simulink library "AFCToolbox2023a"  (R2023a)
settings: Solver=VariableStepAuto  StartTime=0.0  StopTime=10.0  RelTol=1e-3
undefined symbols (not defined in the file or in its folder): AFC5Toolbox_SimuMoudle, AFCToolbox, ax, ay, az, btnSample, C_d, C_dm, C_m, C_t, Control, d, declination_table, dp0, dp1, dp2, dp3, dt, euler_0, g0, I_xyz, inclination_table, J_m, lmd_high, lmd_low, lp_acc_knoise, lp_acc_max, lp_acc_min, lp_acc_seed, lp_GPS_BL_max, lp_GPS_BL_min, lp_GPS_H_max, lp_GPS_H_min, lp_GPS_knoise, lp_GPS_seed, lp_GPS_vel_max, lp_GPS_vel_min, lp_gyro_knoise, lp_gyro_max, lp_gyro_min, lp_gyro_seed, lp_hf_vwind, lp_hs_vwind_interp, lp_kaerorho, lp_kaeroT, lp_kIxyz, lp_kmass, lp_momentx_A0, lp_momentx_Af, lp_momentx_ts, lp_momenty_A0, lp_momenty_Af, lp_momenty_ts, lp_momentz_A0, lp_momentz_Af, lp_momentz_ts, lp_vf_vwind, lp_vs_vwind_interp, lp_vwind_thetax, lp_vwind_thetaz ... (+54)
libraries: $bdroot x104, simulink x75, etargetslib x32, sharedtransform x13, simulink_extras x12, dspstat3 x11, aerolibconvert2 x9, aerolibtransform2 x3, aerolibutil x2, matrix_library x1
(part 5 of 10)

== system AFCToolbox2023a/SimuMoudle/Forces & Moments1/Moments/Disturb ==
  Moment : Inport
  Demux : Demux  Outputs=3
  Dist Mx : Subsystem  mask(Step Disturbe){ts_0=lp_momentx_ts, A0=lp_momentx_A0, Af=lp_momentx_Af}
      mask prompts: ts_0 "Step time (s) :"; A0 "Initial Value (N.m) :"; Af "Final Value (N.m) :"
  Dist My : Subsystem  mask(Step Disturbe){ts_0=lp_momenty_ts, A0=lp_momenty_A0, Af=lp_momenty_Af}
      mask prompts: ts_0 "Step time (s) :"; A0 "Initial Value (N.m) :"; Af "Final Value (N.m) :"
  Dist Mz : Subsystem  mask(Step Disturbe){ts_0=lp_momentz_ts, A0=lp_momentz_A0, Af=lp_momentz_Af}
      mask prompts: ts_0 "Step time (s) :"; A0 "Initial Value (N.m) :"; Af "Final Value (N.m) :"
  Mux : Mux  Inputs=3
  M : Outport
  wires:
  Mux/1 -> M/1
  Moment/1 -> Demux/1
  Demux/1 -> Dist Mx/1(N)
  Demux/2 -> Dist My/1(N)
  Demux/3 -> Dist Mz/1(N)
  Dist Mx/1(D) -> Mux/1
  Dist My/1(D) -> Mux/2
  Dist Mz/1(D) -> Mux/3

== system AFCToolbox2023a/SimuMoudle/Forces & Moments1/Parameters/Air Parameter1 ==
  V : Inport
  h(m) : Inport  Port=2
  Air Model : Subsystem
  Fcn : Fcn  Expr=g0*(6371^2/(6371+u)^2)
  Gain3 : Gain  Gain=0.001
  vel : Scope
  Mach : Outport
  q : Outport  Port=2
  Pressure : Outport  Port=3
  g : Outport  Port=4
  wires:
  Air Model/3(Pressure) -> Pressure/1
  Gain3/1 -> Fcn/1, Air Model/2(h (km))
  Air Model/1(dongYaTou) -> q/1
  Air Model/2(Mach) -> Mach/1
  V/1 -> vel/1, Air Model/1(v)
  h(m)/1 -> Gain3/1
  Fcn/1 -> g/1

== system AFCToolbox2023a/SimuMoudle/Forces & Moments1/Parameters/Inertia Solution ==
  Constant : Constant  Value=I_xyz
  lp_kIxyz : Gain  Gain=lp_kIxyz
  Inertia : Outport
  wires:
  Constant/1 -> lp_kIxyz/1
  lp_kIxyz/1 -> Inertia/1

== system AFCToolbox2023a/SimuMoudle/Forces & Moments1/Parameters/Wind Velocity ==
  height : Inport
  >lp_hf_vwind : Switch  Criteria=u2 > Threshold  Threshold=lp_hf_vwind  SaturateOnIntegerOverflow=off  InputSameDT=off
  Lookup Table h-v wind : Lookup  InputValues=lp_hs_vwind_interp  Table=lp_vs_vwind_interp  SaturateOnIntegerOverflow=off
  Vector : Subsystem
  lp_vf_vwind : Constant  Value=lp_vf_vwind
  lp_vwind_thetax : Constant  Value=lp_vwind_thetax
  lp_vwind_thetaz : Constant  Value=lp_vwind_thetaz
  V Wind : Outport
  wires:
  lp_vf_vwind/1 -> >lp_hf_vwind/1
  height/1 -> Lookup Table h-v wind/1, >lp_hf_vwind/2
  Lookup Table h-v wind/1 -> >lp_hf_vwind/3
  lp_vwind_thetaz/1 -> Vector/2(thetaz)
  lp_vwind_thetax/1 -> Vector/3(thetax)
  Vector/1(xyz) -> V Wind/1
  >lp_hf_vwind/1 -> Vector/1(abs)

== system AFCToolbox2023a/SimuMoudle/Forces & Moments1/Parameters/mass P ==
  Constant 1 : Constant  Value=mass
  lp_kmass : Gain  Gain=lp_kmass
  mass : Outport
  wires:
  lp_kmass/1 -> mass/1
  Constant 1/1 -> lp_kmass/1

== system AFCToolbox2023a/SimuMoudle/Forces & Moments1/Parameters/modulus of vector ==
  vector : Inport
  Divide2 : Product
  Math Function : Math  Operator=sqrt  SignedPower=on
  Sum of Elements : Sum  Inputs=+
  modulus : Outport
  wires:
  Math Function/1 -> modulus/1
  vector/1 -> Divide2/1, Divide2/2
  Divide2/1 -> Sum of Elements/1
  Sum of Elements/1 -> Math Function/1

== system AFCToolbox2023a/SimuMoudle/Position-Control/Consistent formation control /一致性控制——F1 ==
  u0_k : Inport
  X0_k_1 : Inport  Port=2
  X1_k_1 : Inport  Port=3
  X2_k_1 : Inport  Port=4
  dp : Inport  Port=5
  Add{,1..2,4..5,8} (6 alike) : Sum  Inputs=+-
  Add3 : Sum  Inputs=-+
  Add6 : Sum  Inputs=+++
  Add7 : Sum  Inputs=+--
  Bus Selector : BusSelector  OutputSignals=p1_k_1
  Bus Selector1 : BusSelector  OutputSignals=p2_k_1
  Bus Selector2 : BusSelector  OutputSignals=p0_k_1
  Bus Selector3 : BusSelector  OutputSignals=dp1,dp0
  Bus Selector4 : BusSelector  OutputSignals=dp1,dp2
  Bus Selector5 : BusSelector  OutputSignals=v111_k_1
  Bus Selector6 : BusSelector  OutputSignals=v000_k_1
  Demux1 : Demux  Outputs=3
  Gain : Gain  Gain=2
  Gain1 : Gain  Gain=0.5
  Gain2 : Gain  Gain=2
  MATLAB Function1 : MATLAB Function  TreatAsAtomicUnit=on
  MATLAB Function2 : MATLAB Function  TreatAsAtomicUnit=on
  MATLAB Function4 : MATLAB Function  TreatAsAtomicUnit=on
  Mux : Mux  Inputs=3
  Subsystem1 : Subsystem
  X0_k_1_2 : InportShadow  Port=2
  X1_k_1_1 : InportShadow  Port=3
  dp1 : InportShadow  Port=5
  u1_k : Outport
  wires:
  MATLAB Function2/1(result) -> Mux/3
  Demux1/2 -> MATLAB Function1/1(r)
  Demux1/3 -> MATLAB Function2/1(r)
  Demux1/1 -> MATLAB Function4/1(r)
  MATLAB Function1/1(result) -> Mux/2
  MATLAB Function4/1(result) -> Mux/1
  Bus Selector2/1 -> Add/2  "<p0_k_1>"
  dp1/1 -> Bus Selector4/1
  Add8/1 -> u1_k/1
  Gain/1 -> Add6/1
  Add/1 -> Add3/2
  Bus Selector1/1 -> Add1/2  "<p2_k_1>"
  Add5/1 -> Add6/3
  Add2/1 -> Add3/1
  Add4/1 -> Add5/2
  Mux/1 -> Add7/3
  X0_k_1/1 -> Bus Selector6/1
  dp/1 -> Bus Selector3/1
  Subsystem1/1(wxyz) -> Gain/1
  Add1/1 -> Add5/1
  Add7/1 -> Gain2/1
  Bus Selector3/2 -> Add2/2  "<dp0>"
  Bus Selector4/2 -> Add4/2  "<dp2>"
  u0_k/1 -> Add8/1
  Bus Selector3/1 -> Add2/1  "<dp1>"
  X1_k_1/1 -> Bus Selector/1
  Bus Selector6/1 -> Add7/2  "<v000_k_1>"
  Add6/1 -> Gain1/1
  Gain1/1 -> Demux1/1  "控制量z"
  X1_k_1_1/1 -> Bus Selector5/1
  Bus Selector4/1 -> Add4/1  "<dp1>"
  X2_k_1/1 -> Bus Selector1/1
  X0_k_1_2/1 -> Bus Selector2/1
  Bus Selector/1 -> Add1/1, Add/1  "<p1_k_1>"
  Bus Selector5/1 -> Add7/1  "<v111_k_1>"
  Add3/1 -> Add6/2
  Gain2/1 -> Add8/2

== system AFCToolbox2023a/SimuMoudle/Position-Control/Consistent formation control /一致性控制——F2 ==
  dp : Inport
  u0_k : Inport  Port=2
  X0_k_1 : Inport  Port=3
  X1_k_1 : Inport  Port=4
  X2_k_1 : Inport  Port=5
  X3_k_1 : Inport  Port=6
  Add{,1..2,4..5,8} (6 alike) : Sum  Inputs=+-
  Add3 : Sum  Inputs=-+
  Add6 : Sum  Inputs=+++
  Add7 : Sum  Inputs=+--
  Bus Selector : BusSelector  OutputSignals=p1_k_1
  Bus Selector1 : BusSelector  OutputSignals=p2_k_1
  Bus Selector2 : BusSelector  OutputSignals=p2_k_1
  Bus Selector3 : BusSelector  OutputSignals=dp2,dp1
  Bus Selector4 : BusSelector  OutputSignals=dp2,dp3
  Bus Selector5 : BusSelector  OutputSignals=v222_k_1
  Bus Selector6 : BusSelector  OutputSignals=v000_k_1
  Bus Selector7 : BusSelector  OutputSignals=p3_k_1
  Demux1 : Demux  Outputs=3
  Gain : Gain  Gain=2
  Gain1 : Gain  Gain=0.5
  Gain2 : Gain  Gain=2
  MATLAB Function1 : MATLAB Function  TreatAsAtomicUnit=on
  MATLAB Function2 : MATLAB Function  TreatAsAtomicUnit=on
  MATLAB Function3 : MATLAB Function  TreatAsAtomicUnit=on
  Mux : Mux  Inputs=3
  Subsystem2 : Subsystem
  X2_k_1_2 : InportShadow  Port=5
  X2_k_1_3 : InportShadow  Port=5
  dp1 : InportShadow
  u2_k : Outport
  wires:
  MATLAB Function2/1(result) -> Mux/3
  MATLAB Function1/1(result) -> Mux/2
  MATLAB Function3/1(result) -> Mux/1
  Demux1/3 -> MATLAB Function2/1(r)
  Demux1/2 -> MATLAB Function1/1(r)
  Demux1/1 -> MATLAB Function3/1(r)
  Bus Selector4/2 -> Add4/2  "<dp3>"
  Bus Selector3/1 -> Add2/1  "<dp2>"
  Bus Selector7/1 -> Add1/2  "<p3_k_1>"
  X3_k_1/1 -> Bus Selector7/1
  X2_k_1_2/1 -> Bus Selector2/1
  Bus Selector2/1 -> Add1/1  "<p2_k_1>"
  Bus Selector/1 -> Add/2  "<p1_k_1>"
  Bus Selector1/1 -> Add/1  "<p2_k_1>"
  Gain2/1 -> Add8/2
  Add3/1 -> Add6/2
  Bus Selector5/1 -> Add7/1  "<v222_k_1>"
  X2_k_1/1 -> Bus Selector1/1
  Bus Selector4/1 -> Add4/1  "<dp2>"
  X2_k_1_3/1 -> Bus Selector5/1
  Gain1/1 -> Demux1/1  "控制量z"
  Add6/1 -> Gain1/1
  Bus Selector6/1 -> Add7/2  "<v000_k_1>"
  X1_k_1/1 -> Bus Selector/1
  u0_k/1 -> Add8/1
  Bus Selector3/2 -> Add2/2  "<dp1>"
  Add7/1 -> Gain2/1
  Add1/1 -> Add5/1
  Subsystem2/1(wxyz) -> Gain/1
  dp/1 -> Bus Selector3/1
  X0_k_1/1 -> Bus Selector6/1
  Mux/1 -> Add7/3
  Add4/1 -> Add5/2
  Add2/1 -> Add3/1
  Add5/1 -> Add6/3
  Add/1 -> Add3/2
  Gain/1 -> Add6/1
  Add8/1 -> u2_k/1
  dp1/1 -> Bus Selector4/1

== system AFCToolbox2023a/SimuMoudle/Position-Control/Consistent formation control /一致性控制——F3 ==
  dp : Inport
  u0_k : Inport  Port=2
  X0_k_1 : Inport  Port=3
  X1_k_1 : Inport  Port=4
  X2_k_1 : Inport  Port=5
  X3_k_1 : Inport  Port=6
  Add{,1..2,4..5,8} (6 alike) : Sum  Inputs=+-
  Add3 : Sum  Inputs=-+
  Add6 : Sum  Inputs=+++
  Add7 : Sum  Inputs=+--
  Bus Selector : BusSelector  OutputSignals=p2_k_1
  Bus Selector1 : BusSelector  OutputSignals=p3_k_1
  Bus Selector2 : BusSelector  OutputSignals=p3_k_1
  Bus Selector3 : BusSelector  OutputSignals=dp3,dp2
  Bus Selector4 : BusSelector  OutputSignals=dp3,dp1
  Bus Selector5 : BusSelector  OutputSignals=v333_k_1
  Bus Selector6 : BusSelector  OutputSignals=v000_k_1
  Bus Selector7 : BusSelector  OutputSignals=p1_k_1
  Demux1 : Demux  Outputs=3
  Gain : Gain  Gain=2
  Gain1 : Gain  Gain=0.5
  Gain2 : Gain  Gain=2
  MATLAB Function1 : MATLAB Function  TreatAsAtomicUnit=on
  MATLAB Function2 : MATLAB Function  TreatAsAtomicUnit=on
  MATLAB Function3 : MATLAB Function  TreatAsAtomicUnit=on
  Mux : Mux  Inputs=3
  Subsystem1 : Subsystem
  X3_k_1_2 : InportShadow  Port=6
  X3_k_1_3 : InportShadow  Port=6
  dp1 : InportShadow
  u3_k : Outport
  wires:
  MATLAB Function2/1(result) -> Mux/3
  Demux1/2 -> MATLAB Function1/1(r)
  Demux1/3 -> MATLAB Function2/1(r)
  Demux1/1 -> MATLAB Function3/1(r)
  MATLAB Function1/1(result) -> Mux/2
  MATLAB Function3/1(result) -> Mux/1
  Subsystem1/1(wxyz) -> Gain/1
  Bus Selector4/2 -> Add4/2  "<dp1>"
  Bus Selector4/1 -> Add4/1  "<dp3>"
  Bus Selector3/2 -> Add2/2  "<dp2>"
  Bus Selector3/1 -> Add2/1  "<dp3>"
  X1_k_1/1 -> Bus Selector7/1
  X2_k_1/1 -> Bus Selector/1
  X3_k_1/1 -> Bus Selector1/1
  dp1/1 -> Bus Selector4/1
  Add8/1 -> u3_k/1
  Gain/1 -> Add6/1
  Add/1 -> Add3/2
  Add5/1 -> Add6/3
  Add2/1 -> Add3/1
  Add4/1 -> Add5/2
  Mux/1 -> Add7/3
  X0_k_1/1 -> Bus Selector6/1
  dp/1 -> Bus Selector3/1
  Add1/1 -> Add5/1
  Add7/1 -> Gain2/1
  u0_k/1 -> Add8/1
  Bus Selector6/1 -> Add7/2  "<v000_k_1>"
  Add6/1 -> Gain1/1
  Gain1/1 -> Demux1/1  "控制量z"
  X3_k_1_3/1 -> Bus Selector5/1
  Bus Selector5/1 -> Add7/1  "<v333_k_1>"
  Add3/1 -> Add6/2
  Gain2/1 -> Add8/2
  Bus Selector1/1 -> Add/1  "<p3_k_1>"
  Bus Selector/1 -> Add/2  "<p2_k_1>"
  Bus Selector2/1 -> Add1/1  "<p3_k_1>"
  X3_k_1_2/1 -> Bus Selector2/1
  Bus Selector7/1 -> Add1/2  "<p1_k_1>"

== system AFCToolbox2023a/SimuMoudle/Position-Control/Leader/Subsystem ==
  Follower1 : Subsystem
  Follower2 : Subsystem
  Follower3 : Subsystem
  tag scope: X1_k_1=global, X2_k_1=global, X3_k_1=global
  wires:
  Follower3/1(p3_k) -> [p3_k]
  Follower3/4(w3_k) -> [w3_k]
  Follower1/3(v1_k) -> [v1_k]
  Follower2/4(w2_k) -> [w2_k]
  Follower1/1(p1_k) -> [p1_k]
  Follower1/2(X1_k_1) -> [X1_k_1]
  [u] -> Follower3/2(u3_k), Follower2/2(u2_k), Follower1/2(u1_k)
  Follower3/3(v3_k) -> [v3_k]
  Follower1/4(w1_k) -> [w1_k]
  Follower1/5(W1_k) -> [W1_k]
  Follower3/5(W3_k) -> [W3_k]
  Follower2/5(W2_k) -> [W2_k]
  Follower2/3(v2_k) -> [v2_k]
  Follower2/2(X2_k_1) -> [X2_k_1]
  Follower2/1(p2_k) -> [p2_k]
  Follower3/2(X3_k_1) -> [X3_k_1]
  [X0_k_1] -> Follower1/1(X0_k_1), Follower2/1(X0_k_1), Follower3/1(X0_k_1)

== system AFCToolbox2023a/SimuMoudle/Position-Control/Leader/W0-Φ ==
  Digital Clock : DigitalClock  SampleTime=dt
  Gain1 : Gain  Gain=0.2
  Gain2 : Gain  Gain=0.1
  Sin : Trigonometry  Operator=cos
  W0 : Outport
  wires:
  Gain2/1 -> W0/1
  Sin/1 -> Gain2/1
  Gain1/1 -> Sin/1
  Digital Clock/1 -> Gain1/1

== system AFCToolbox2023a/SimuMoudle/Position-Control/Leader/r0-v ==
  Digital Clock : DigitalClock  SampleTime=dt
  Gain1 : Gain  Gain=0.4
  Gain2 : Gain  Gain=0.1
  Scope : Scope
  Sin : Trigonometry
  r0 : Outport
  wires:
  Gain2/1 -> r0/1, Scope/1
  Sin/1 -> Gain2/1
  Gain1/1 -> Sin/1
  Digital Clock/1 -> Gain1/1

== system AFCToolbox2023a/SimuMoudle/Position-Control/Leader/w0-θ ==
  Digital Clock : DigitalClock  SampleTime=dt
  Gain1 : Gain  Gain=0.2
  Gain2 : Gain  Gain=0.1
  Sin : Trigonometry  Operator=cos
  w0 : Outport
  wires:
  Digital Clock/1 -> Gain1/1
  Gain1/1 -> Sin/1
  Sin/1 -> Gain2/1
  Gain2/1 -> w0/1

== system AFCToolbox2023a/SimuMoudle/Position-Control/Leader/质心运动方程 ==
  theta0 : Inport
  phi0 : Inport  Port=2
  v0 : Inport  Port=3
  Cos : Trigonometry  Operator=cos
  Cos1 : Trigonometry  Operator=cos
  Mux : Mux  Inputs=3
  Product : Product  Inputs=3
  Product1 : Product  Inputs=3
  Product2 : Product
  Sin : Trigonometry
  Sin1 : Trigonometry
  v000 : Outport
  wires:
  Sin1/1 -> Product2/1
  Mux/1 -> v000/1
  Product2/1 -> Mux/3
  Cos1/1 -> Product/2, Product1/2
  Sin/1 -> Product1/1
  Product1/1 -> Mux/2
  Product/1 -> Mux/1
  v0/1 -> Product/3, Product1/3, Product2/2
  Cos/1 -> Product/1
  phi0/1 -> Cos1/1, Sin1/1
  theta0/1 -> Sin/1, Cos/1

== system AFCToolbox2023a/SimuMoudle/SimuBaro/Baro model/bias & noise z ==
  normal : Inport
  Sum1 : Sum  Inputs=|++
  Uniform Random Number : UniformRandomNumber  Minimum=noise_min  Maximum=noise_max  Seed=noise_seed  SampleTime=lp_GPS_sample_time
  noise_k : Gain  Gain=noise_k
  real : Outport
  wires:
  noise_k/1 -> Sum1/2
  Uniform Random Number/1 -> noise_k/1
  normal/1 -> Sum1/1
  Sum1/1 -> real/1

== system AFCToolbox2023a/SimuMoudle/SimuGps/LLA model/Subsystem1 ==
  note: 北天东
  note: B:纬度
      | L:经度
      | lat:纬度
      | lon:经度
  X : Inport
  Y : Inport  Port=2
  Z : Inport  Port=3
  Angle Conversion1 : aerolibconvert2/Angle Conversion  IU=rad  OU=deg
  Angle Conversion2 : aerolibconvert2/Angle Conversion  IU=rad  OU=deg
  Bus Creator : BusCreator  Inputs=3
  Bus Creator1 : BusCreator  Inputs=3
  Display5 : Display
  ECEF地心坐标系-经纬高 : MATLAB Function  TreatAsAtomicUnit=on
  LLA2NED : Subsystem
  Mux1 : Mux  Inputs=3
  Mux2 : Mux  Inputs=3
  Mux4 : Mux  Inputs=3
  Scope : Scope
  Scope1 : Scope
  Scope2 : Scope  NumInputPorts=2
  command word1 : Constant  Value=1.978927027963337
  command word10 : Constant  Value=0.402497166193948
  command word11 : Constant  Value=500
  command word3 : Constant  Value=0.402497166193948
  command word4 : Constant  Value=500
  command word9 : Constant  Value=1.978927027963337
  北天东-ECEF地心坐标系 : MATLAB Function  TreatAsAtomicUnit=on
  LLA : Outport
  wires:
  Mux2/1 -> LLA/1
  [lbn] -> LLA2NED/2(LLA)
  X/1 -> Mux4/1, 北天东-ECEF地心坐标系/1(pn)
  Angle Conversion1/1 -> Bus Creator/2  "lat"
  Angle Conversion2/1 -> Bus Creator/1  "lon"
  Mux4/1 -> Scope2/1
  ECEF地心坐标系-经纬高/2(b) -> Bus Creator1/1, Mux2/1  "lat"
  command word9/1 -> Angle Conversion2/1  "lon"
  ECEF地心坐标系-经纬高/1(l) -> Bus Creator1/2, Mux2/2  "lon"
  Bus Creator/1 -> LLA2NED/1(LLA0)
  Bus Creator1/1 -> [lbn], Display5/1, Scope1/1
  LLA2NED/1("sensorout ") -> Scope2/2
  ECEF地心坐标系-经纬高/3(h) -> Bus Creator1/3, Mux2/3  "alt"
  command word10/1 -> Angle Conversion1/1  "lat"
  command word11/1 -> Bus Creator/3  "alt"
  Z/1 -> Mux4/3, 北天东-ECEF地心坐标系/3(pe)
  Y/1 -> Mux4/2, 北天东-ECEF地心坐标系/2(ph)
  Mux1/1 -> Scope/1
  command word4/1 -> 北天东-ECEF地心坐标系/6(Alt0)
  command word3/1 -> 北天东-ECEF地心坐标系/5(Lat0)
  command word1/1 -> 北天东-ECEF地心坐标系/4(Lon0)
  北天东-ECEF地心坐标系/3(DZ) -> ECEF地心坐标系-经纬高/3(z), Mux1/3
  北天东-ECEF地心坐标系/2(DY) -> ECEF地心坐标系-经纬高/2(y), Mux1/2
  北天东-ECEF地心坐标系/1(DX) -> ECEF地心坐标系-经纬高/1(x), Mux1/1

== system AFCToolbox2023a/SimuMoudle/SimuGps/LLA model/bias & noise x ==
  normal : Inport
  Sum1 : Sum  Inputs=|++
  Uniform Random Number : UniformRandomNumber  Minimum=noise_min  Maximum=noise_max  Seed=noise_seed  SampleTime=lp_GPS_sample_time
  noise_k : Gain  Gain=noise_k
  real : Outport
  wires:
  Sum1/1 -> real/1
  normal/1 -> Sum1/1
  Uniform Random Number/1 -> noise_k/1
  noise_k/1 -> Sum1/2

== system AFCToolbox2023a/SimuMoudle/SimuGps/LLA model/bias & noise x2 ==
  normal : Inport
  Sum1 : Sum  Inputs=|++
  Uniform Random Number : UniformRandomNumber  Minimum=noise_min  Maximum=noise_max  Seed=noise_seed  SampleTime=lp_GPS_sample_time
  noise_k : Gain  Gain=noise_k
  real : Outport
  wires:
  noise_k/1 -> Sum1/2
  Uniform Random Number/1 -> noise_k/1
  normal/1 -> Sum1/1
  Sum1/1 -> real/1

== system AFCToolbox2023a/SimuMoudle/SimuGps/LLA model/bias & noise z ==
  normal : Inport
  Sum1 : Sum  Inputs=|++
  Uniform Random Number : UniformRandomNumber  Minimum=noise_min  Maximum=noise_max  Seed=noise_seed  SampleTime=lp_GPS_sample_time
  noise_k : Gain  Gain=noise_k
  real : Outport
  wires:
  Sum1/1 -> real/1
  normal/1 -> Sum1/1
  Uniform Random Number/1 -> noise_k/1
  noise_k/1 -> Sum1/2

== system AFCToolbox2023a/SimuMoudle/SimuGps/Vel model/bias & noise x ==
  normal : Inport
  Sum1 : Sum  Inputs=|++
  Uniform Random Number : UniformRandomNumber  Minimum=noise_min  Maximum=noise_max  Seed=noise_seed  SampleTime=lp_GPS_sample_time
  noise_k : Gain  Gain=noise_k
  real : Outport
  wires:
  noise_k/1 -> Sum1/2
  Uniform Random Number/1 -> noise_k/1
  normal/1 -> Sum1/1
  Sum1/1 -> real/1

== system AFCToolbox2023a/SimuMoudle/SimuGps/Vel model/bias & noise x1 ==
  normal : Inport
  Sum1 : Sum  Inputs=|++
  Uniform Random Number : UniformRandomNumber  Minimum=noise_min  Maximum=noise_max  Seed=noise_seed  SampleTime=lp_GPS_sample_time
  noise_k : Gain  Gain=noise_k
  real : Outport
  wires:
  noise_k/1 -> Sum1/2
  Uniform Random Number/1 -> noise_k/1
  normal/1 -> Sum1/1
  Sum1/1 -> real/1

== system AFCToolbox2023a/SimuMoudle/SimuGps/Vel model/bias & noise x3 ==
  normal : Inport
  Sum1 : Sum  Inputs=|++
  Uniform Random Number : UniformRandomNumber  Minimum=noise_min  Maximum=noise_max  Seed=noise_seed  SampleTime=lp_GPS_sample_time
  noise_k : Gain  Gain=noise_k
  real : Outport
  wires:
  Sum1/1 -> real/1
  normal/1 -> Sum1/1
  Uniform Random Number/1 -> noise_k/1
  noise_k/1 -> Sum1/2

== system AFCToolbox2023a/SimuMoudle/SimuICM/acclerate  model2/Subsystem ==
  normal : Inport
  Add4 : Sum
  Add5 : Sum
  Constant5 : Constant  Value=0
  Constant8 : Constant  Value=dt
  Delay1 : Delay  DelayLength=1  InitialConditionSource=Input port
      settings: InputPortMap=u0,p4
  Display1 : Display
  GM均方根 : Constant  Value=100*10e-6
  GM时间常数 : Constant  Value=3600
  MATLAB Function : MATLAB Function  TreatAsAtomicUnit=on
  Scope5 : Scope
  Scope6 : Scope  NumInputPorts=2
  bias & noise x1 : Subsystem  mask(Bias and Noise Model){noise_min=lp_acc_min, noise_max=lp_acc_max, noise_seed=lp_acc_seed, noise_k=lp_acc_knoise}
      mask prompts: noise_min "Minimum of the noise:"; noise_max "Maximum of the noise:"; noise_seed "Seed of the noise:"; noise_k "Noise coefficiet:"
  white noise : RandomNumber  Variance=100*10e-6*g0  SampleTime=lp_sample_time
  real : Outport
  wires:
  GM均方根/1 -> MATLAB Function/3(accNoiseStdDev)
  GM时间常数/1 -> MATLAB Function/2(correlationTimeConstant)
  Constant5/1 -> Delay1/2
  Delay1/1 -> MATLAB Function/1(accBias)
  Constant8/1 -> MATLAB Function/4(dt)
  MATLAB Function/1(accData) -> bias & noise x1/1(GM), Scope5/1, Delay1/1
  white noise/1 -> Add4/1
  bias & noise x1/1(real) -> Add4/2
  Add5/1 -> Display1/1, Scope6/2, real/1
  normal/1 -> Scope6/1, Add5/1
  Add4/1 -> Add5/2

== system AFCToolbox2023a/SimuMoudle/SimuICM/acclerate  model2/Subsystem1 ==
  normal : Inport
  Add4 : Sum
  Add5 : Sum
  Constant5 : Constant  Value=0
  Constant8 : Constant  Value=dt
  Delay1 : Delay  DelayLength=1  InitialConditionSource=Input port
      settings: InputPortMap=u0,p4
  Display1 : Display
  GM均方根 : Constant  Value=100*10e-6
  GM时间常数 : Constant  Value=3600
  MATLAB Function : MATLAB Function  TreatAsAtomicUnit=on
  Scope5 : Scope
  Scope6 : Scope  NumInputPorts=2
  bias & noise x1 : Subsystem  mask(Bias and Noise Model){noise_min=lp_acc_min, noise_max=lp_acc_max, noise_seed=lp_acc_seed, noise_k=lp_acc_knoise}
      mask prompts: noise_min "Minimum of the noise:"; noise_max "Maximum of the noise:"; noise_seed "Seed of the noise:"; noise_k "Noise coefficiet:"
  white noise : RandomNumber  Variance=100*10e-6*g0  SampleTime=lp_sample_time
  real : Outport
  wires:
  Add4/1 -> Add5/2
  normal/1 -> Add5/1, Scope6/1
  Add5/1 -> real/1, Scope6/2, Display1/1
  bias & noise x1/1(real) -> Add4/2
  white noise/1 -> Add4/1
  MATLAB Function/1(accData) -> Delay1/1, Scope5/1, bias & noise x1/1(GM)
  Constant8/1 -> MATLAB Function/4(dt)
  Delay1/1 -> MATLAB Function/1(accBias)
  Constant5/1 -> Delay1/2
  GM时间常数/1 -> MATLAB Function/2(correlationTimeConstant)
  GM均方根/1 -> MATLAB Function/3(accNoiseStdDev)

== system AFCToolbox2023a/SimuMoudle/SimuICM/acclerate  model2/Subsystem2 ==
  normal : Inport
  Add4 : Sum
  Add5 : Sum
  Constant5 : Constant  Value=0
  Constant8 : Constant  Value=dt
  Delay1 : Delay  DelayLength=1  InitialConditionSource=Input port
      settings: InputPortMap=u0,p4
  Display1 : Display
  GM均方根 : Constant  Value=100*10e-6
  GM时间常数 : Constant  Value=3600
  MATLAB Function : MATLAB Function  TreatAsAtomicUnit=on
  Scope5 : Scope
  Scope6 : Scope  NumInputPorts=2
  bias & noise x1 : Subsystem  mask(Bias and Noise Model){noise_min=lp_acc_min, noise_max=lp_acc_max, noise_seed=lp_acc_seed, noise_k=lp_acc_knoise}
      mask prompts: noise_min "Minimum of the noise:"; noise_max "Maximum of the noise:"; noise_seed "Seed of the noise:"; noise_k "Noise coefficiet:"
  white noise : RandomNumber  Variance=100*10e-6*g0  SampleTime=lp_sample_time
  real : Outport
  wires:
  GM均方根/1 -> MATLAB Function/3(accNoiseStdDev)
  GM时间常数/1 -> MATLAB Function/2(correlationTimeConstant)
  Constant5/1 -> Delay1/2
  Delay1/1 -> MATLAB Function/1(accBias)
  Constant8/1 -> MATLAB Function/4(dt)
  MATLAB Function/1(accData) -> bias & noise x1/1(GM), Scope5/1, Delay1/1
  white noise/1 -> Add4/1
  bias & noise x1/1(real) -> Add4/2
  Add5/1 -> Display1/1, Scope6/2, real/1
  normal/1 -> Scope6/1, Add5/1
  Add4/1 -> Add5/2

== system AFCToolbox2023a/SimuMoudle/SimuICM/acclerate  model2/bias & noise x ==
  normal : Inport
  Display : Display
  Scope : Scope
  Scope1 : Scope
  Scope2 : Scope
  Sum1 : Sum  Inputs=|++
  Uniform Random Number : UniformRandomNumber  Minimum=noise_min  Maximum=noise_max  Seed=noise_seed  SampleTime=lp_sample_time
  noise_k : Gain  Gain=noise_k
  real : Outport
  wires:
  Sum1/1 -> Display/1, Scope2/1, real/1
  normal/1 -> Sum1/1
  noise_k/1 -> Sum1/2, Scope/1
  Uniform Random Number/1 -> Scope1/1, noise_k/1

== system AFCToolbox2023a/SimuMoudle/SimuICM/acclerate  model2/bias & noise y ==
  normal : Inport
  Sum1 : Sum  Inputs=|++
  Uniform Random Number : UniformRandomNumber  Minimum=noise_min  Maximum=noise_max  Seed=noise_seed  SampleTime=lp_sample_time
  noise_k : Gain  Gain=noise_k
  real : Outport
  wires:
  noise_k/1 -> Sum1/2
  Uniform Random Number/1 -> noise_k/1
  normal/1 -> Sum1/1
  Sum1/1 -> real/1

== system AFCToolbox2023a/SimuMoudle/SimuICM/acclerate  model2/bias & noise z ==
  normal : Inport
  Sum1 : Sum  Inputs=|++
  Uniform Random Number : UniformRandomNumber  Minimum=noise_min  Maximum=noise_max  Seed=noise_seed  SampleTime=lp_sample_time
  noise_k : Gain  Gain=noise_k
  real : Outport
  wires:
  Sum1/1 -> real/1
  normal/1 -> Sum1/1
  Uniform Random Number/1 -> noise_k/1
  noise_k/1 -> Sum1/2

== system AFCToolbox2023a/SimuMoudle/SimuICM/gyro model1/Subsystem ==
  normal : Inport
  Add4 : Sum
  Add5 : Sum
  Constant5 : Constant  Value=0
  Constant6 : Constant  Value=3600
  Constant7 : Constant  Value=0.1
  Constant8 : Constant  Value=dt
  Delay1 : Delay  DelayLength=1  InitialConditionSource=Input port
      settings: InputPortMap=u0,p4
  Display1 : Display
  MATLAB Function : MATLAB Function  TreatAsAtomicUnit=on
  Scope5 : Scope
  Scope6 : Scope
  bias & noise x1 : Subsystem  mask(Bias and Noise Model){noise_min=lp_gyro_min, noise_max=lp_gyro_max, noise_seed=lp_gyro_seed, noise_k=lp_gyro_knoise}
      mask prompts: noise_min "Minimum of the noise:"; noise_max "Maximum of the noise:"; noise_seed "Seed of the noise:"; noise_k "Noise coefficiet:"
  white noise : RandomNumber  Variance=0.01*pi/(180*3600)  SampleTime=lp_sample_time
  real : Outport
  wires:
  Add4/1 -> Add5/2
  normal/1 -> Add5/1
  Add5/1 -> real/1, Scope6/1, Display1/1
  bias & noise x1/1(real) -> Add4/2
  white noise/1 -> Add4/1
  MATLAB Function/1(gyroData) -> Delay1/1, Scope5/1, bias & noise x1/1(GM)
  Constant8/1 -> MATLAB Function/4(dt)
  Delay1/1 -> MATLAB Function/1(gyroBias)
  Constant5/1 -> Delay1/2
  Constant6/1 -> MATLAB Function/2(correlationTimeConstant)
  Constant7/1 -> MATLAB Function/3(gyroNoiseStdDev)

== system AFCToolbox2023a/SimuMoudle/SimuICM/gyro model1/Subsystem1 ==
  normal : Inport
  Add4 : Sum
  Add5 : Sum
  Constant5 : Constant  Value=0
  Constant6 : Constant  Value=3600
  Constant7 : Constant  Value=0.1
  Constant8 : Constant  Value=dt
  Delay1 : Delay  DelayLength=1  InitialConditionSource=Input port
      settings: InputPortMap=u0,p4
  Display1 : Display
  MATLAB Function : MATLAB Function  TreatAsAtomicUnit=on
  Scope5 : Scope
  Scope6 : Scope
  bias & noise x1 : Subsystem  mask(Bias and Noise Model){noise_min=lp_gyro_min, noise_max=lp_gyro_max, noise_seed=lp_gyro_seed, noise_k=lp_gyro_knoise}
      mask prompts: noise_min "Minimum of the noise:"; noise_max "Maximum of the noise:"; noise_seed "Seed of the noise:"; noise_k "Noise coefficiet:"
  white noise : RandomNumber  Variance=0.01*pi/(180*3600)  SampleTime=lp_sample_time
  real : Outport
  wires:
  Constant7/1 -> MATLAB Function/3(gyroNoiseStdDev)
  Constant6/1 -> MATLAB Function/2(correlationTimeConstant)
  Constant5/1 -> Delay1/2
  Delay1/1 -> MATLAB Function/1(gyroBias)
  Constant8/1 -> MATLAB Function/4(dt)
  MATLAB Function/1(gyroData) -> bias & noise x1/1(GM), Scope5/1, Delay1/1
  white noise/1 -> Add4/1
  bias & noise x1/1(real) -> Add4/2
  Add5/1 -> Display1/1, Scope6/1, real/1
  normal/1 -> Add5/1
  Add4/1 -> Add5/2

== system AFCToolbox2023a/SimuMoudle/SimuICM/gyro model1/Subsystem2 ==
  normal : Inport
  Add4 : Sum
  Add5 : Sum
  Constant5 : Constant  Value=0
  Constant6 : Constant  Value=3600
  Constant7 : Constant  Value=0.1
  Constant8 : Constant  Value=dt
  Delay1 : Delay  DelayLength=1  InitialConditionSource=Input port
      settings: InputPortMap=u0,p4
  Display1 : Display
  MATLAB Function : MATLAB Function  TreatAsAtomicUnit=on
  Scope5 : Scope
  Scope6 : Scope
  bias & noise x1 : Subsystem  mask(Bias and Noise Model){noise_min=lp_gyro_min, noise_max=lp_gyro_max, noise_seed=lp_gyro_seed, noise_k=lp_gyro_knoise}
      mask prompts: noise_min "Minimum of the noise:"; noise_max "Maximum of the noise:"; noise_seed "Seed of the noise:"; noise_k "Noise coefficiet:"
  white noise : RandomNumber  Variance=0.01*pi/(180*3600)  SampleTime=lp_sample_time
  real : Outport
  wires:
  Add4/1 -> Add5/2
  normal/1 -> Add5/1
  Add5/1 -> real/1, Scope6/1, Display1/1
  bias & noise x1/1(real) -> Add4/2
  white noise/1 -> Add4/1
  MATLAB Function/1(gyroData) -> Delay1/1, Scope5/1, bias & noise x1/1(GM)
  Constant8/1 -> MATLAB Function/4(dt)
  Delay1/1 -> MATLAB Function/1(gyroBias)
  Constant5/1 -> Delay1/2
  Constant6/1 -> MATLAB Function/2(correlationTimeConstant)
  Constant7/1 -> MATLAB Function/3(gyroNoiseStdDev)

== system AFCToolbox2023a/SimuMoudle/SimuICM/gyro model1/bias & noise x ==
  normal : Inport
  Display : Display
  Scope : Scope
  Scope1 : Scope
  Scope2 : Scope
  Sum1 : Sum  Inputs=|++
  Uniform Random Number : UniformRandomNumber  Minimum=noise_min  Maximum=noise_max  Seed=noise_seed  SampleTime=lp_sample_time
  noise_k : Gain  Gain=noise_k
  real : Outport
  wires:
  Uniform Random Number/1 -> noise_k/1, Scope1/1
  noise_k/1 -> Scope/1, Sum1/2
  normal/1 -> Sum1/1
  Sum1/1 -> real/1, Scope2/1, Display/1

== system AFCToolbox2023a/SimuMoudle/SimuICM/gyro model1/bias & noise y ==
  normal : Inport
  Sum1 : Sum  Inputs=|++
  Uniform Random Number : UniformRandomNumber  Minimum=noise_min  Maximum=noise_max  Seed=noise_seed  SampleTime=lp_sample_time
  noise_k : Gain  Gain=noise_k
  real : Outport
  wires:
  Sum1/1 -> real/1
  normal/1 -> Sum1/1
  Uniform Random Number/1 -> noise_k/1
  noise_k/1 -> Sum1/2

== system AFCToolbox2023a/SimuMoudle/SimuICM/gyro model1/bias & noise z ==
  normal : Inport
  Sum1 : Sum  Inputs=|++
  Uniform Random Number : UniformRandomNumber  Minimum=noise_min  Maximum=noise_max  Seed=noise_seed  SampleTime=lp_sample_time
  noise_k : Gain  Gain=noise_k
  real : Outport
  wires:
  noise_k/1 -> Sum1/2
  Uniform Random Number/1 -> noise_k/1
  normal/1 -> Sum1/1
  Sum1/1 -> real/1

== system AFCToolbox2023a/SimuMoudle/UAV/Equations of Motion/NED2LLA ==
  lat(deg) : Inport
  lon(deg) : Inport  Port=2
  h(m) : Inport  Port=3
  N : Inport  Port=4
  U : Inport  Port=5
  E : Inport  Port=6
  Add : Sum
  Demux : Demux  Outputs=2
  Direction Cosine Matrix ECEF to NED : aerolibtransform2/Direction Cosine Matrix ECEF to NED
  ECEF Position to LLA1 : ECEF2LLA  R=6378137
  Gain : Gain  Gain=-1
  LLA to ECEF Position : LLA2ECEF  R=6378137
  Mux : Mux  Inputs=2
  Mux1 : Mux  Inputs=3
  Product : Product  Multiplication=Matrix(*)
  Transpose : Math  Operator=transpose  SignedPower=on
  latout(deg) : Outport
  lonout(deg) : Outport  Port=2
  altout(m) : Outport  Port=3
  wires:
  LLA to ECEF Position/1 -> Add/1
  Transpose/1 -> Product/1
  Direction Cosine Matrix ECEF to NED/1 -> Transpose/1
  h(m)/1 -> LLA to ECEF Position/2
  Add/1 -> ECEF Position to LLA1/1
  Product/1 -> Add/2
  ECEF Position to LLA1/2 -> altout(m)/1
  lat(deg)/1 -> Mux/1
  lon(deg)/1 -> Mux/2
  Mux/1 -> Direction Cosine Matrix ECEF to NED/1, LLA to ECEF Position/1
  ECEF Position to LLA1/1 -> Demux/1
  Demux/1 -> latout(deg)/1
  Demux/2 -> lonout(deg)/1
  U/1 -> Gain/1
  N/1 -> Mux1/1
  E/1 -> Mux1/2
  Gain/1 -> Mux1/3
  Mux1/1 -> Product/2

== system AFCToolbox2023a/SimuMoudle/UAV/Equations of Motion/w x ( I w ) ==
  a(1) a(2) a(3) : Inport
  b(1) b(2) b(3) : Inport  Port=2
  Product : Product  RndMeth=Zero
  Product1 : Product  RndMeth=Zero
  Selector : Selector  InputPortWidth=3  IndexOptions=Index vector (dialog)  Indices=[2 3 1]  OutputSizes=1
  Selector1 : Selector  InputPortWidth=3  IndexOptions=Index vector (dialog)  Indices=[3 1 2]  OutputSizes=1
  Selector2 : Selector  InputPortWidth=3  IndexOptions=Index vector (dialog)  Indices=[3 1 2]  OutputSizes=1
  Selector3 : Selector  InputPortWidth=3  IndexOptions=Index vector (dialog)  Indices=[2 3 1]  OutputSizes=1
  Sum : Sum  Inputs=+|-
  c(1) c(2) c(3) : Outport
  wires:
  b(1) b(2) b(3)/1 -> Selector2/1, Selector3/1
  a(1) a(2) a(3)/1 -> Selector1/1, Selector/1
  Selector2/1 -> Product/2
  Selector1/1 -> Product1/1
  Selector3/1 -> Product1/2
  Selector/1 -> Product/1
  Sum/1 -> c(1) c(2) c(3)/1
  Product1/1 -> Sum/2
  Product/1 -> Sum/1

== system AFCToolbox2023a/SimuMoudle/UAV/Forces & Moments/Forces ==
  B to G : Inport
  w1234 : Inport  Port=2
  Vb_a : Inport  Port=3
  mass : Inport  Port=4
  g : Inport  Port=5
  Abs : Abs  SaturateOnIntegerOverflow=off
  Constant 0 : Constant  Value=0
  Constant 1 : Constant  Value=0
  Gain : Gain  Gain=C_t
  Gain1 : Gain  Gain=C_d
  Gain2 : Gain  Gain=-1
  Mux : Mux  Inputs=3
  N SD : Scope  Commented=on
  Product B2G * F : Product  Multiplication=Matrix(*)  RndMeth=Zero
  Product F/G : Product  Inputs=*/  RndMeth=Zero
  Product mg0 : Product  Inputs=**  RndMeth=Zero
  Product mgxyz : Product  Inputs=**  RndMeth=Zero
  Product1 : Product
  Product2 : Product
  Scope : Scope
  Subsystem : Subsystem
  Sum of Elements : Sum  Inputs=+
  add : Sum  Inputs=2
  add1 : Sum  Inputs=2
  "F " : Outport
  wires:
  Vb_a/1 -> Abs/1, Product2/1
  B to G/1 -> Product B2G * F/1
  Product mgxyz/1 -> add1/2
  add1/1 -> "F "/1
  Product B2G * F/1 -> add1/1
  Product F/G/1 -> N SD/1
  g/1 -> Subsystem/2(g0), Product mg0/2
  mass/1 -> Product mgxyz/1, Product mg0/1
  Subsystem/1(gravity) -> Product mgxyz/2
  Constant 0/1 -> Subsystem/1(Zero)
  Product mg0/1 -> Product F/G/2
  w1234/1 -> Product1/2, Product1/1
  Product1/1 -> Sum of Elements/1
  Sum of Elements/1 -> Gain/1
  Abs/1 -> Product2/2
  Product2/1 -> Gain1/1
  Gain/1 -> Gain2/1
  Constant 1/1 -> Mux/2, Mux/1
  Mux/1 -> add/1
  add/1 -> Scope/1, Product B2G * F/2, Product F/G/1
  Gain2/1 -> Mux/3
  Gain1/1 -> add/2

== system AFCToolbox2023a/SimuMoudle/UAV/Forces & Moments/Moments ==
  w_xyz1 : Inport
  w_1234 : Inport  Port=2
  Abs : Abs  SaturateOnIntegerOverflow=off
  Constant : Constant  Value=[1 -1 -1 1;1 1 -1 -1]
  Constant1 : Constant  Value=[1 -1 1 -1]
  Constant2 : Constant  Value=[1 -1 1 -1]
  Constant3 : Constant  Value=[-1 1 -1 1]
  Constant4 : Constant  Value=0
  Disturb : Subsystem
  Dot Product : DotProduct  OutDataTypeStr=Inherit: Inherit via internal rule
  Dot Product1 : DotProduct  OutDataTypeStr=Inherit: Inherit via internal rule
  Dot Product2 : DotProduct  OutDataTypeStr=Inherit: Inherit via internal rule
  Gain : Gain  Gain=C_t
  Gain1 : Gain  Gain=d
  Gain2 : Gain  Gain=C_m
  Gain3 : Gain  Gain=C_dm
  Gain4 : Gain  Gain=-1
  Gain5 : Gain  Gain=J_m
  Gain6 : Gain  Gain=sqrt(2)/2
  M1 : Scope
  Mux : Mux  Inputs=2
  Mux1 : Mux  Inputs=3
  Product : Product  Multiplication=Matrix(*)
  Product{1,3,6..7} (4 alike) : Product
  Scope : Scope
  Selector : Selector  InputPortWidth=3  IndexOptions=Index vector (dialog)  Indices=2  OutputSizes=1
  Selector1 : Selector  InputPortWidth=3  IndexOptions=Index vector (dialog)  Indices=1  OutputSizes=1
  Subtract : Sum  Inputs=3
  Sum of Elements : Sum  Inputs=+
  Sum of Elements1 : Sum  Inputs=+
  M : Outport
  wires:
  Subtract/1 -> Disturb/1(Moment)
  Disturb/1(M) -> M/1, M1/1
  Product1/1 -> Gain2/1, Gain/1
  Gain/1 -> Gain1/1
  Constant/1 -> Gain6/1
  Gain1/1 -> Product/2
  Gain2/1 -> Dot Product2/2
  Constant1/1 -> Dot Product2/1
  Product/1 -> Mux/1
  Dot Product2/1 -> Mux/2
  Abs/1 -> Product3/2
  Product3/1 -> Gain3/1
  w_xyz1/1 -> Abs/1, Product3/1, Selector/1, Selector1/1
  Gain3/1 -> Gain4/1
  Constant2/1 -> Dot Product/1
  Constant3/1 -> Dot Product1/1
  Selector/1 -> Product6/2
  Dot Product/1 -> Sum of Elements/1
  Sum of Elements/1 -> Product6/1
  Dot Product1/1 -> Sum of Elements1/1
  Selector1/1 -> Product7/2
  Sum of Elements1/1 -> Product7/1
  Product6/1 -> Mux1/1
  Product7/1 -> Mux1/2
  Constant4/1 -> Mux1/3
  Mux1/1 -> Gain5/1
  Gain4/1 -> Subtract/1
  Mux/1 -> Subtract/2
  Gain6/1 -> Product/1
  w_1234/1 -> Scope/1, Product1/2, Product1/1, Dot Product1/2, Dot Product/2
  Gain5/1 -> Subtract/3

== system AFCToolbox2023a/SimuMoudle/UAV/Forces & Moments/Parameters ==
  V_xyz : Inport
  xyz : Inport  Port=2
  B to G : Inport  Port=3
  Air Parameter1 : Subsystem
  Gain : Gain  Gain=-1
  Inertia Solution : Subsystem
  Math Function : Math  Operator=transpose  SignedPower=on
  Product : Product  Multiplication=Matrix(*)
  Selector : Selector  InputPortWidth=3  IndexOptions=Index vector (dialog)  Indices=3  OutputSizes=1
  Sum : Sum  Inputs=|+-
  Terminator1 : Terminator
  Terminator2 : Terminator
  Terminator3 : Terminator
  Wind Velocity : Subsystem
  mass P : Subsystem
  modulus of vector : Subsystem  mask(modulus of vector){}
      mask help: solve the modulus of a vector |v|
      mask Display: fprintf('Vector\nModulus')
  Vb_a : Outport
  mass : Outport  Port=2
  Inertia : Outport  Port=3
  g : Outport  Port=4
  wires:
  V_xyz/1 -> Sum/1
  xyz/1 -> Selector/1
  modulus of vector/1(modulus) -> Air Parameter1/1(V)
  Selector/1 -> Air Parameter1/2(h(m)), Wind Velocity/1(height)
  Inertia Solution/1(Inertia) -> Inertia/1
  Wind Velocity/1(V Wind) -> Sum/2
  Sum/1 -> Gain/1, modulus of vector/1(vector)
  Air Parameter1/1(Mach) -> Terminator2/1
  mass P/1(mass) -> mass/1
  Air Parameter1/2(q) -> Terminator1/1
  Air Parameter1/3(Pressure) -> Terminator3/1
  B to G/1 -> Math Function/1
  Math Function/1 -> Product/1
  Product/1 -> Vb_a/1
  Gain/1 -> Product/2
  Air Parameter1/4(g) -> g/1

== system AFCToolbox2023a/SimuMoudle/UAV/Forces & Moments/acc_body ==
  B2G : Inport
  g : Inport  Port=2
  acc_no_g : Inport  Port=3
  Add : Sum
  Constant : Constant  Value=0
  Gain : Gain  Gain=-1
  Mux : Mux  Inputs=3
  Product : Product  Multiplication=Matrix(*)
  Transpose : Math  Operator=transpose  SignedPower=on
  acc : Outport
  wires:
  Gain/1 -> Mux/3
  acc_no_g/1 -> Add/2
  Constant/1 -> Mux/2, Mux/1
  B2G/1 -> Transpose/1
  g/1 -> Gain/1
  Mux/1 -> Add/1
  Add/1 -> Product/2
  Transpose/1 -> Product/1
  Product/1 -> acc/1

== system AFCToolbox2023a/基础导航算法模型库/ECL EKF/Bias Eliminate2/Subsystem ==
  data : Inport
  Buffer : Buffer  N=50  V=49  OutputFrames=off
  Buffer1 : Buffer  N=50  V=49  OutputFrames=off
  Buffer2 : Buffer  N=50  V=49  OutputFrames=off
  Demux : Demux  Outputs=3
  Mean4 : dspstat3/Mean  run=off  reset_popup=None  directionMode=Entire input  dimension=3  roiEnable=off  roiType=Rectangles  roiPortion=Entire ROI  roiOutput=Individual statistics for each ROI  roiFlag=off  roundingMode=Floor  overflowMode=off  outputDataTypeStr=Inherit: Same as accumulator  outputMin=[]  outputMax=[]  outputLastDataTypeStr=Inherit: Same as accumulator
  Mean5 : dspstat3/Mean  run=off  reset_popup=None  directionMode=Entire input  dimension=3  roiEnable=off  roiType=Rectangles  roiPortion=Entire ROI  roiOutput=Individual statistics for each ROI  roiFlag=off  roundingMode=Floor  overflowMode=off  outputDataTypeStr=Inherit: Same as accumulator  outputMin=[]  outputMax=[]  outputLastDataTypeStr=Inherit: Same as accumulator
  Mean6 : dspstat3/Mean  run=off  reset_popup=None  directionMode=Entire input  dimension=3  roiEnable=off  roiType=Rectangles  roiPortion=Entire ROI  roiOutput=Individual statistics for each ROI  roiFlag=off  roundingMode=Floor  overflowMode=off  outputDataTypeStr=Inherit: Same as accumulator  outputMin=[]  outputMax=[]  outputLastDataTypeStr=Inherit: Same as accumulator
  Scope : Scope  NumInputPorts=2
  Vector Concatenate : Concatenate  NumInputs=3
  mean_data : Outport
  wires:
  Mean6/1 -> Vector Concatenate/3
  Demux/2 -> Buffer1/1
  Buffer/1 -> Mean4/1  "fbx_buff"
  Mean5/1 -> Vector Concatenate/2
  Buffer2/1 -> Mean6/1  "fbz_buff"
  Demux/1 -> Buffer/1
  Buffer1/1 -> Mean5/1  "fby_buff"
  Demux/3 -> Buffer2/1
  Mean4/1 -> Vector Concatenate/1
  Vector Concatenate/1 -> Scope/2, mean_data/1
  data/1 -> Scope/1, Demux/1

== system AFCToolbox2023a/基础导航算法模型库/ECL EKF/Subsystem/GPS Fusion1 ==
  note: control.cpp -> controlGpsFusion(...) ->
      | gps_control.cpp -> updateGpsVel(...) -> updateGpsPos（...) -> fuseGpsVel( -> fuseGpsPos)
  "states " : Inport
  meas_pos : Inport  Port=2
  meas_vel : Inport  Port=3
  gps_alt_ref : Inport  Port=4
  meas_Hgt : Inport  Port=5
  baro_hgt_offset : Inport  Port=6
  "P " : Inport  Port=7
  Enable : EnablePort
  Constant : Constant  Value=gpspos_innov_gate
  Constant1 : Constant  Value=gpsvel_innov_gate
  Constant2 : Constant  Value=gpsvel_obsvar
  Constant3 : Constant  Value=gpspos_obsvar
  Control BARO_Hgt Fusion : Subsystem
  Control GPS_Pos Fusion1 : MATLAB Function  TreatAsAtomicUnit=on
  Control GPS_Vel Fusion1 : MATLAB Function  TreatAsAtomicUnit=on
  Data Type Conversion{1..6} (6 alike) : DataTypeConversion  OutDataTypeStr=single  SaturateOnIntegerOverflow=off  RndMeth=Floor
  Logical Operator : Logic  Operator=NOT  AllPortsSameDT=off  OutDataTypeStr=boolean
  Reshape : Reshape
  Switch1 : Switch  Threshold=1  OutDataTypeStr=single  SaturateOnIntegerOverflow=off  InputSameDT=off
  Switch2 : Switch  Threshold=1  OutDataTypeStr=single  SaturateOnIntegerOverflow=off  InputSameDT=off
  Terminator{,1..3} (4 alike) : Terminator
  gps_hgt_offset : Constant  Value=0
  gps_z_flag : Constant  Value=baro_z_flag
  gps_z_flag1 : Constant  Value=baro_z_flag
  states : Outport
  P : Outport  Port=2
  wires:
  Logical Operator/1 -> Switch2/2, Switch1/2
  gps_z_flag1/1 -> Logical Operator/1
  Control BARO_Hgt Fusion/2(P) -> Switch2/3
  Control BARO_Hgt Fusion/1(states) -> Switch1/3
  Switch2/1 -> P/1
  Switch1/1 -> states/1
  Data Type Conversion5/1 -> Control GPS_Pos Fusion1/4(innov_gate)
  Data Type Conversion4/1 -> Control GPS_Pos Fusion1/5(obs_var)
  Data Type Conversion3/1 -> Control GPS_Pos Fusion1/6(contrl_GPSflag)
  Data Type Conversion2/1 -> Control GPS_Pos Fusion1/8(gps_hgt_offset)
  Data Type Conversion6/1 -> Control GPS_Vel Fusion1/4(innov_gate)
  Data Type Conversion1/1 -> Control GPS_Vel Fusion1/5(obs_var)
  Constant1/1 -> Data Type Conversion6/1
  Control GPS_Pos Fusion1/2(P) -> Control BARO_Hgt Fusion/2("P "), Switch2/1
  Control GPS_Pos Fusion1/1(states) -> Control BARO_Hgt Fusion/1("states "), Switch1/1
  Control GPS_Vel Fusion1/2(P) -> Control GPS_Pos Fusion1/2("P ")
  Control GPS_Vel Fusion1/1(states) -> Control GPS_Pos Fusion1/1("states ")
  "P "/1 -> Control GPS_Vel Fusion1/2("P ")  "P"
  "states "/1 -> Control GPS_Vel Fusion1/1("states ")
  gps_alt_ref/1 -> Control GPS_Pos Fusion1/7(gps_alt_ref)
  meas_Hgt/1 -> Control BARO_Hgt Fusion/3(meas_Hgt)
  Control GPS_Vel Fusion1/4(innov_var) -> Terminator1/1
  meas_pos/1 -> Control GPS_Pos Fusion1/3(measPos)
  Control GPS_Pos Fusion1/3(innovation) -> Terminator3/1
  Constant/1 -> Data Type Conversion5/1
  gps_z_flag/1 -> Data Type Conversion3/1
  Reshape/1 -> Data Type Conversion1/1
  Constant2/1 -> Reshape/1
  baro_hgt_offset/1 -> Control BARO_Hgt Fusion/4(baro_hgt_offset)
  meas_vel/1 -> Control GPS_Vel Fusion1/3(measVel)
  gps_hgt_offset/1 -> Data Type Conversion2/1
  Constant3/1 -> Data Type Conversion4/1
  Control GPS_Vel Fusion1/3(innovation) -> Terminator/1
  Control GPS_Pos Fusion1/4(innov_var) -> Terminator2/1

== system AFCToolbox2023a/基础导航算法模型库/ECL EKF/Subsystem/Mag Fusion ==
  "states " : Inport
  "P " : Inport  Port=2
  meas_Mag : Inport  Port=3
  measDec : Inport  Port=4
  Control MagDeclination Fusion1 : MATLAB Function  TreatAsAtomicUnit=on
  Control Magneto meter Fusion2 : MATLAB Function  TreatAsAtomicUnit=on
  params.mag_noise1 : Constant  Value=R_MAG^2  OutDataTypeStr=single
  params.mag_noise2 : Constant  Value=R_decl  OutDataTypeStr=single
  flag : Outport
  states : Outport  Port=2
  P : Outport  Port=3
  wires:
  params.mag_noise2/1 -> Control MagDeclination Fusion1/3(R_decl)
  Control MagDeclination Fusion1/2(P) -> P/1
  Control MagDeclination Fusion1/1(states) -> states/1
  "P "/1 -> Control Magneto meter Fusion2/2("P ")  "P"
  Control Magneto meter Fusion2/1(fault_status_flags_bad_mag) -> flag/1
  Control Magneto meter Fusion2/3(P) -> Control MagDeclination Fusion1/2("P ")
  "states "/1 -> Control Magneto meter Fusion2/1("states ")
  Control Magneto meter Fusion2/2(states) -> Control MagDeclination Fusion1/1("states ")
  measDec/1 -> Control MagDeclination Fusion1/4(measDec)
  meas_Mag/1 -> Control Magneto meter Fusion2/3(Measmag)
  params.mag_noise1/1 -> Control Magneto meter Fusion2/4(R_MAG)

== system AFCToolbox2023a/基础导航算法模型库/ECL EKF/Subsystem/Subsystem2 ==
  imu_delta_angle : Inport
  imu_delta_vel : Inport  Port=2
  "states " : Inport  Port=3
  lat : Inport  Port=4
  "P " : Inport  Port=5
  Constant : Constant  Value=dt  OutDataTypeStr=single
  Constant2 : Constant  Value=zeros(1,3)  OutDataTypeStr=single
  Predict Covariance : MATLAB Function  TreatAsAtomicUnit=on
  Predict States : MATLAB Function  TreatAsAtomicUnit=on
  Scope1 : Scope
  Scope2 : Scope
  Selector1 : Selector  InputPortWidth=24  IndexOptions=Index vector (dialog)  Indices=[1 2 3 4]  OutputSizes=1
  states : Outport
  P : Outport  Port=2
  wires:
  Constant/1 -> Predict Covariance/5(dt), Predict States/4(dt)
  Selector1/1 -> Scope2/1
  Predict States/1(corrected_delta_ang) -> Predict Covariance/1(delta_ang)
  Predict States/2(corrected_delta_vel) -> Predict Covariance/2(delta_vel)
  imu_delta_vel/1 -> Scope1/1, Predict States/3(delta_vel)
  "states "/1 -> Selector1/1, Predict States/1("states ")
  Predict States/3(states) -> Predict Covariance/3(states), states/1
  imu_delta_angle/1 -> Predict States/2(delta_ang)
  Constant2/1 -> Predict Covariance/6(accel_bias_inhibit)
  Predict Covariance/1(P) -> P/1
  lat/1 -> Predict States/5(latitude)
  "P "/1 -> Predict Covariance/4("P ")

== system AFCToolbox2023a/基础导航算法模型库/ECL EKF/init_state/ALIGN TILT 1 ==
  note: ekf.cpp -> initialseTilt()
  initAccel : Inport
  Constant : Constant
  Constant1 : Constant  Value=0
  Constant2 : Constant
  Dot Product : DotProduct  OutDataTypeStr=Inherit: Inherit via internal rule
  Logical Operator : Logic  AllPortsSameDT=off  OutDataTypeStr=boolean
  Scope : Scope
  Sqrt : Sqrt
  Subsystem : Subsystem
  Sum of Elements : Sum  Inputs=+
  Switch1 : Switch  Criteria=u2 > Threshold  Threshold=5  SaturateOnIntegerOverflow=off  InputSameDT=off
  Switch2 : Switch  Threshold=14  SaturateOnIntegerOverflow=off  InputSameDT=off
  Switch3 : Switch  Threshold=1  SaturateOnIntegerOverflow=off  InputSameDT=off
  init_quat : Constant  Value=[1;0;0;0]  OutDataTypeStr=single
  state(1:4) : Outport
  wires:
  Sum of Elements/1 -> Sqrt/1
  Constant/1 -> Switch1/1
  Switch2/1 -> Logical Operator/2
  Sqrt/1 -> Switch2/2, Switch1/2
  Constant1/1 -> Switch2/1, Switch1/3
  init_quat/1 -> Switch3/3, Subsystem/1(init_quat)
  Switch1/1 -> Logical Operator/1
  Dot Product/1 -> Sum of Elements/1
  Constant2/1 -> Switch2/3
  initAccel/1 -> Subsystem/2(initAccel), Dot Product/2, Dot Product/1
  Subsystem/1(quat) -> Switch3/1
  Logical Operator/1 -> Switch3/2
  Switch3/1 -> Scope/1, state(1:4)/1

== system AFCToolbox2023a/基础导航算法模型库/ECL EKF/init_state/InitState_accel1 ==
  imu_data_del_vel : Inport
  Constant1 : Constant
  Constant2 : Constant  Value=0
  Detect Increase1 : simulink/Logic and Bit Operations/Detect Increase  vinit=0.0  OutDataTypeStr=boolean
  Digital Clock : DigitalClock  SampleTime=-1
  Gain : Gain  Gain=1/dt
  Memory : Memory  InheritSampleTime=on
  Scope{,1..3} (4 alike) : Scope
  Subsystem : Subsystem
  Switch : Switch  Criteria=u2 > Threshold  Threshold=10  SaturateOnIntegerOverflow=off  InputSameDT=off
  Switch2 : Switch  Threshold=1  SaturateOnIntegerOverflow=off  InputSameDT=off
  initAccel1 : MATLAB Function  Commented=on  TreatAsAtomicUnit=on
  initaccel : Outport
  wires:
  imu_data_del_vel/1 -> Scope1/1, Subsystem/1(data)
  Subsystem/1(mean_data) -> Scope2/1, Memory/1, Gain/1, Switch2/1
  Gain/1 -> Scope/1, initaccel/1
  Detect Increase1/1 -> Scope3/1, Switch2/2
  Constant2/1 -> Switch/3
  Digital Clock/1 -> Switch/2
  Switch/1 -> Detect Increase1/1
  Constant1/1 -> Switch/1
  Memory/1 -> Switch2/3

== system AFCToolbox2023a/基础导航算法模型库/ECL EKF/init_state/InitState_baro1 ==
  note: VehicleAirData.cpp -> PressureToAltitude(...)
  baro_data_Pa : Inport
  states : Inport  Port=2
  QGC_sensor_reinit : Inport  Port=3
  imu_delta_ang : Inport  Port=4
  Bus Creator : BusCreator  Inputs=2
  Data Type Conversion6 : DataTypeConversion  OutDataTypeStr=single  SaturateOnIntegerOverflow=off  RndMeth=Floor
  Gain : Gain  Gain=-1
  Gain1 : Gain  Gain=-1
  Gain2 : Gain  Gain=-1
  MATLAB Function : MATLAB Function  TreatAsAtomicUnit=on
  Reshape : Reshape  OutputDimensionality=Customize  OutputDimensions=[3,1]
  Reshape1 : Reshape  OutputDimensionality=Customize  OutputDimensions=[4,1]
  Reshape2 : Reshape  OutputDimensionality=Customize  OutputDimensions=[2,1]
  Scope1 : Scope  NumInputPorts=2
  Scope2 : Scope
  Scope3 : Scope
  Scope6 : Scope  NumInputPorts=2
  Scope7 : Scope
  Selector : Selector  InputPortWidth=24  IndexOptions=Index vector (dialog)  Indices=[1,2,3,4]  OutputSizes=1
  Selector1 : Selector  InputPortWidth=24  IndexOptions=Index vector (dialog)  Indices=[5:7]  OutputSizes=1
  Selector2 : Selector  InputPortWidth=24  IndexOptions=Index vector (dialog)  Indices=[23,24]  OutputSizes=1
  Sum : Sum  Inputs=|+-
  TD_baro : Subsystem
  compensateBaroForDynamicPressure : MATLAB Function  TreatAsAtomicUnit=on
  reinit_baro0 : Subsystem
  BARO_Data : Outport
  wires:
  baro_data_Pa/1 -> MATLAB Function/1(pressure_pa)
  Selector/1 -> Reshape1/1  "quaternion"
  Selector1/1 -> Reshape/1  "vel"
  Selector2/1 -> Reshape2/1  "wind_vel"
  MATLAB Function/1(altitude) -> Data Type Conversion6/1, compensateBaroForDynamicPressure/1(baro_alt_uncompensated)
  states/1 -> Selector2/1, Selector1/1, Selector/1
  imu_delta_ang/1 -> compensateBaroForDynamicPressure/5(delta_ang)
  Reshape/1 -> compensateBaroForDynamicPressure/3(output_new_vel)
  Reshape1/1 -> compensateBaroForDynamicPressure/2(output_quaternion)
  Reshape2/1 -> compensateBaroForDynamicPressure/4(state_wind_vel)
  reinit_baro0/1(dataout) -> Sum/2, Bus Creator/2, Scope7/1  "init_barohgt"
  Bus Creator/1 -> BARO_Data/1
  Sum/1 -> Scope2/1, Bus Creator/1  "Baro_hgt"
  Gain/1 -> reinit_baro0/1(Data), Scope1/1
  compensateBaroForDynamicPressure/1(baro_sample_new) -> Gain1/1
  Gain1/1 -> Scope1/2, Scope3/1
  QGC_sensor_reinit/1 -> reinit_baro0/2(QGC_sensor_reinit)
  Data Type Conversion6/1 -> Gain/1, Scope6/1, TD_baro/1(H_baro)
  TD_baro/2(H_baro_TD) -> Gain2/1  "H_baro_m_TD"
  Gain2/1 -> Scope6/2, Sum/1
